simulink model "Fourier"  (Simulink 7.7)
settings: Solver=ode45  SolverMode=SingleTasking  StartTime=0.0  StopTime=T  MaxStep=1e-3  RelTol=1e-3  AbsTol=1e-6
values from neighbouring files (symbols this model uses):
  A = 2    [Base_main.m]    (also in Base_otima_ini.m; Fourier_main.m)
  DC = 50    [Base_main.m]    (also in Base_otima_ini.m; Fourier_main.m)
  n = 1    [Base_main.m]    (also in Base_otima_ini.m; exercicio_01.m = linspace(N_neg,N_pos,N); exercicio_02.m = linspace(N_neg,N_pos,N))
  T = 1.0    (= 1)    [Base_main.m]    (also in Base_otima_ini.m; Fourier_main.m)
settings Model: Creator=vanderleiparro  LastModifiedBy=vanderleiparro
settings DataIOCC: LimitDataPoints=off  SignalLoggingName=sigsOut
settings OptimizationCC: BooleanDataType=off
settings DebuggingCC: SaveWithParameterizedLinksMsg=none  SignalResolutionControl=TryResolveAllWithWarning  SolverPrmCheckMsg=none  MultiTaskDSMMsg=warning  MultiTaskCondExecSysMsg=none  StrictBusMsg=None
settings HardwareCC: TargetUnknown=on
settings RTWCC: IncludeERTFirstTime=on

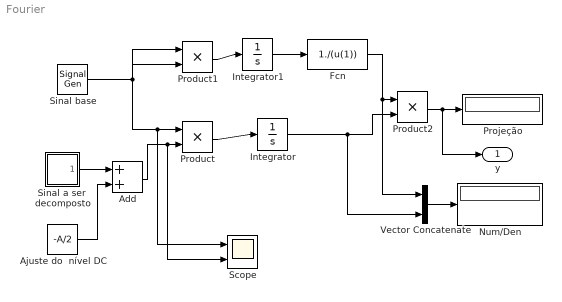
== system Fourier ==
  Add : Sum
  Ajuste do  nível DC : Constant  Value=-A/2
  Fcn : Fcn  Expr=1./(u(1))
  Integrator : Integrator
  Integrator1 : Integrator
  Num/Den : Display
      settings: Format=short_e
  Product : Product  SaturateOnIntegerOverflow=on  InputSameDT=on  OutDataTypeStr=Inherit: Same as first input
  Product1 : Product  SaturateOnIntegerOverflow=on  InputSameDT=on  OutDataTypeStr=Inherit: Same as first input
  Product2 : Product  SaturateOnIntegerOverflow=on  InputSameDT=on  OutDataTypeStr=Inherit: Same as first input
  Projeção : Display
      settings: Format=short_e
  Scope : Scope  NumInputPorts=2
      settings: YMin=-5~-5  YMax=5~5
  Sinal a ser  decomposto : Subsystem  mask(Pulse Generator){period=T, duty=DC, amplitude=A, start=0}
      mask prompts: period "Period (secs):"; duty "Duty cycle (% of period):"; start "Start time:"
      mask help: Pulse Generator
      mask Help: Pulse generator which ensures pulse transitions are hit. Provides a vector of pulses when the height is entered as a vector.  Unmask to see how it works.
      mask Display: plot(0,0,100,100,[95,90,90,75,75,60,60,45,45,30,30,15,15,5],[25,25,75,75,25,25,75,75,25,25,75,75,25,25]);
  Sinal base : SignalGenerator  Frequency=n*inv(T)
  Vector Concatenate : Concatenate  Mode=Multidimensional array
  y : Outport
  wires:
  Product/1 -> Integrator/1
  Sinal base/1 -> Product1/2, Product/1, Scope/1, Product1/1
  Product1/1 -> Integrator1/1
  Integrator1/1 -> Fcn/1
  Fcn/1 -> Product2/1, Vector Concatenate/1
  Integrator/1 -> Product2/2, Vector Concatenate/2
  Product2/1 -> Projeção/1, y/1
  Sinal a ser  decomposto/1(out1) -> Add/1
  Add/1 -> Product/2, Scope/2
  Ajuste do  nível DC/1 -> Add/2
  Vector Concatenate/1 -> Num/Den/1

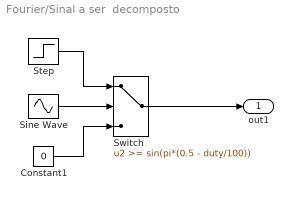
== system Fourier/Sinal a ser  decomposto ==
  Constant1 : Constant  Value=0
  Sine Wave : Sin  Frequency=2*pi./period  Phase=-2*pi*(start./period + duty/200 - 1/4)
  Step : Step  Time=start  After=amplitude
  Switch : Switch  Threshold=sin(pi*(0.5 - duty/100))  SaturateOnIntegerOverflow=on  InputSameDT=on
  out1 : Outport  InitialOutput=0
  wires:
  Sine Wave/1 -> Switch/2
  Switch/1 -> out1/1
  Constant1/1 -> Switch/3
  Step/1 -> Switch/1
